simulink model "tst4"  (R2024b)
settings: Solver=ode45  StartTime=0.0  StopTime=100  FixedStep=0.1  RelTol=1e-3  EnableMultiTasking=on
Description:
  | Simulating Automatic Climate Control Systems
  | 
  | This example shows how to use Simulink(R) and Stateflow(R) to simulate the working of
  | an automatic climate control system in a car. You can enter a temperature
  | value you would like the air in the car to reach by double clicking the
  | User Setpoint in Celsius Block and entering the temperature value. You can
  | also set the External Temperature in Celsius in a similar way. The
  | numerical display on the right-hand side of the model shows the reading
  | of a temperature sensor placed behind the driver's head. This is the
  | temperature that the driver should be feeling. When the model is run and
  | the climate control is active, it is this display box whose value changes
  | to show the change of temperature in the car.
settings Model: ModifiedByFormat=The MathWorks, Inc.  Creator=The MathWorks, Inc.  LastModifiedBy=The MathWorks, Inc.
settings SolverCC: AlgebraicLoopSolver=TrustRegion  MaxZcPerStep=1
settings DataIOCC: LimitDataPoints=on  SaveFormat=Array  ReturnWorkspaceOutputs=off  SignalLoggingName=sigsOut
settings OptimizationCC: ReuseModelBlockBuffer=off  ExpressionDepthLimit=2147483647  InitFltsAndDblsToZero=on  LifeSpan=inf
settings DebuggingCC: SaveWithParameterizedLinksMsg=none  SignalResolutionControl=TryResolveAllWithWarning  MultiTaskDSMMsg=warning  MultiTaskCondExecSysMsg=none  SigSpecEnsureSampleTimeMsg=none  FcnCallInpInsideContextMsg=warning  UnconnectedInputMsg=warning  UnconnectedOutputMsg=warning  UnconnectedLineMsg=warning  StateNameClashWarn=warning  SFUnexpectedBacktrackingDiag=warning  SFNoUnconditionalDefaultTransitionDiag=warning  SFExecutionAtInitializationDiag=none  ArithmeticOperatorsInVariantConditions=warning
settings HardwareCC: ProdBitPerPointer=32  ProdBitPerSizeT=32  ProdBitPerPtrDiffT=32  ProdLargestAtomicFloat=None  ProdIntDivRoundTo=Undefined  ProdEndianess=Unspecified  ProdWordSize=32  ProdHWDeviceType=32-bit Generic
settings ModelReferenceCC: EnableRefExpFcnMdlSchedulingChecks=on  PropagateSignalLabelsOutOfModel=off
settings SFSimCC: SimUseLocalCustomCode=off  SimParseCustomCode=off  CustomCodeUndefinedFunction=UseInterfaceOnly
settings RTWCC: RTWUseLocalCustomCode=off  GPUComputeCapability=3.5  DLArmComputeVersion=19.05
settings CodeAppCC: StateflowObjectComments=on
settings GRTTargetCC: TargetFcnLib=ansi_tfl_tmw.mat  TargetLangStandard=C89/C90 (ANSI)  CombineOutputUpdateFcns=off  GRTInterface=on
settings ConfigComp: CovMetricSettings=dw  CovSaveCumulativeToWorkspaceVar=on  CovSaveSingleToWorkspaceVar=on  CovExternalEMLEnable=off  CovSFcnEnable=off

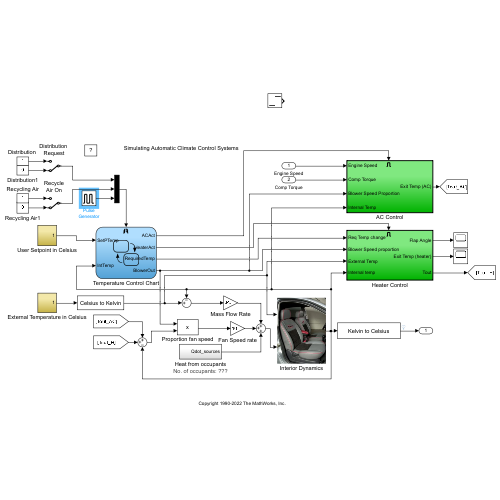
[thumbnail: Simulink's stored preview of the top-level diagram]
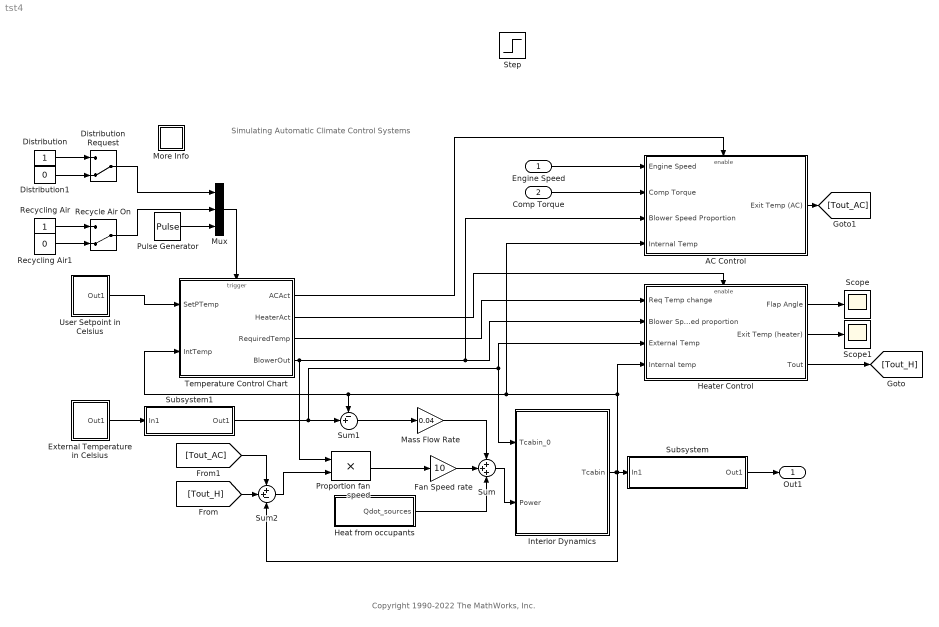
== system tst4 ==
  note: Simulating Automatic Climate Control Systems
  note: Copyright 1990-2022 The MathWorks, Inc.
  Engine Speed : Inport
  Comp Torque : Inport  Port=2
  AC Control : Subsystem  TreatAsAtomicUnit=on
  "Distribution " : Constant
  Distribution Request : ManualSwitch  CurrentSetting=0
  "Distribution1 " : Constant  Value=0
  External Temperature in Celsius : Subsystem
  Fan Speed rate : Gain  Gain=10  SaturateOnIntegerOverflow=on  OutDataTypeStr=Inherit: Same as input  ParamDataTypeStr=Inherit: Same as input
  Heat from occupants : Subsystem
      settings: AttributesFormatString=No. of occupants: %<N>
  Heater Control : Subsystem  TreatAsAtomicUnit=on
  Interior Dynamics : Subsystem  mask(Vehicle Cabin Dynamics){}
      mask Display: image('$imagefile'); % Use "Edit Image" on toolstrip to change.
  Mass Flow Rate : Gain  Gain=0.04  SaturateOnIntegerOverflow=on  OutDataTypeStr=Inherit: Same as input  ParamDataTypeStr=Inherit: Same as input
  More Info : Subsystem
      settings: OpenFcn=showExample('simulink_automotive/SimulatingAutomaticClimateControlSystemsExample')
      mask Display: disp('?')
  Mux : Mux  Inputs=3
  Proportion fan speed : Product  InputSameDT=on  SaturateOnIntegerOverflow=on  OutDataTypeStr=Inherit: Same as first input
  Pulse Generator : DiscretePulseGenerator  PulseType=Time based  Period=1/60  PulseWidth=50
  Recycle Air On : ManualSwitch  CurrentSetting=0
  Recycling Air : Constant
  Recycling Air1 : Constant  Value=0
  Scope : Scope
  Scope1 : Scope
  Step : Step  SampleTime=0
  Subsystem : Subsystem
      mask Display: disp('Kelvin to Celsius')
  Subsystem1 : Subsystem
      mask Display: disp('Celsius to Kelvin')
  Sum : Sum  Inputs=+++  InputSameDT=on  SaturateOnIntegerOverflow=on  OutDataTypeStr=Inherit: Same as first input
  Sum1 : Sum  Inputs=-+|  InputSameDT=on  SaturateOnIntegerOverflow=on  OutDataTypeStr=Inherit: Same as first input
  Sum2 : Sum  Inputs=++-  InputSameDT=on  SaturateOnIntegerOverflow=on  OutDataTypeStr=Inherit: Same as first input
  Temperature Control Chart : Stateflow chart  TreatAsAtomicUnit=on
  User Setpoint in Celsius : Subsystem
  Out1 : Outport
  wires:
  "Distribution "/1 -> Distribution Request/1
  "Distribution1 "/1 -> Distribution Request/2
  Recycling Air1/1 -> Recycle Air On/2
  User Setpoint in Celsius/1(Out1) -> Temperature Control Chart/1(SetPTemp)
  Recycling Air/1 -> Recycle Air On/1
  Interior Dynamics/1("Tcabin ") -> Sum2/3, Heater Control/4(Internal temp), AC Control/4(Internal Temp), Sum1/1, Temperature Control Chart/2(IntTemp), Subsystem/1(In1)
  Subsystem/1(Out1) -> Out1/1
  External Temperature in Celsius/1(Out1) -> Subsystem1/1(In1)
  Mass Flow Rate/1 -> Sum/1
  Sum1/1 -> Mass Flow Rate/1
  Subsystem1/1(Out1) -> Sum1/2, Interior Dynamics/1(Tcabin_0), Heater Control/3(External Temp)
  Sum2/1 -> Proportion fan speed/2
  Temperature Control Chart/4(BlowerOut) -> AC Control/3(Blower Speed Proportion), Heater Control/2(Blower Speed proportion), Proportion fan speed/1
  Proportion fan speed/1 -> Fan Speed rate/1
  Temperature Control Chart/2(" HeaterAct") -> Heater Control/Enable
  Heater Control/3(Tout) -> [Tout_H]
  [Tout_H] -> Sum2/2
  Temperature Control Chart/1(" ACAct") -> AC Control/Enable
  [Tout_AC] -> Sum2/1
  Temperature Control Chart/3(RequiredTemp) -> Heater Control/1(Req Temp change)
  AC Control/1(Exit Temp (AC)) -> [Tout_AC]
  Mux/1 -> Temperature Control Chart/Trigger
  Sum/1 -> Interior Dynamics/2(Power)
  Recycle Air On/1 -> Mux/2
  Distribution Request/1 -> Mux/1
  Fan Speed rate/1 -> Sum/2
  Heat from occupants/1(Qdot_sources) -> Sum/3
  Heater Control/1(Flap Angle) -> Scope/1
  Heater Control/2(Exit Temp (heater)) -> Scope1/1
  Engine Speed/1 -> AC Control/1(Engine Speed)
  Comp Torque/1 -> AC Control/2(Comp Torque)
  Pulse Generator/1 -> Mux/3

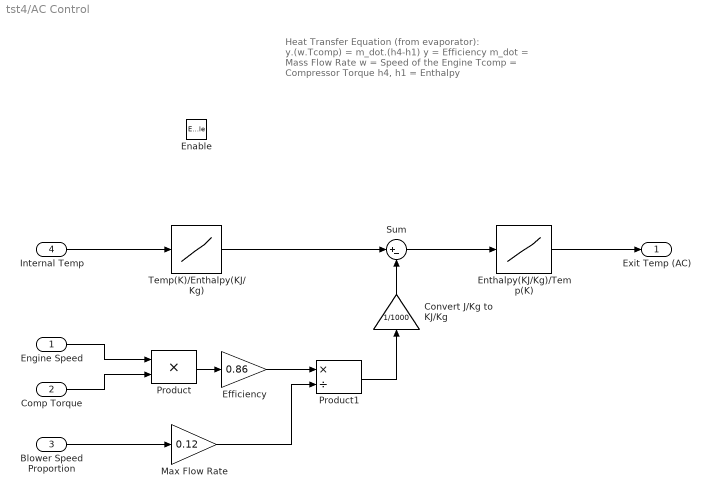
== system tst4/AC Control ==
  note: Heat Transfer Equation (from evaporator):
      |
      | y.(w.Tcomp) = m_dot.(h4-h1)
      |
      |          y = Efficiency
      |  m_dot = Mass Flow Rate
      | 	  w = Speed of the Engine
      | Tcomp = Compressor Torque
      |  h4, h1 = Enthalpy
  Engine Speed : Inport
  Comp Torque : Inport  Port=2
  Blower Speed Proportion : Inport  Port=3
  Internal Temp : Inport  Port=4
  Enable : EnablePort  StatesWhenEnabling=reset  PropagateVarSize=During execution  ZeroCross=off
  Convert J/Kg to KJ/Kg : Gain  Gain=1/1000
  Efficiency : Gain  Gain=0.86  SaturateOnIntegerOverflow=on  OutDataTypeStr=Inherit: Same as input  ParamDataTypeStr=Inherit: Same as input
  Enthalpy(KJ/Kg)/Temp(K) : Lookup_n-D  NumberOfTableDimensions=1  BreakpointsForDimension1=[ 219.97 230.02 240.02 250.05 260.09 270.11 280.13 285.14 290.16 295.17 300.19 305.22 310.24 315.27 320.29]  Table=[220 230 240 250 260 270 280 285 290 295 300 305 310 315 320]  SaturateOnIntegerOverflow=on
  Max Flow Rate : Gain  Gain=0.12  SaturateOnIntegerOverflow=on  OutDataTypeStr=Inherit: Same as input  ParamDataTypeStr=Inherit: Same as input
  Product : Product  InputSameDT=on  SaturateOnIntegerOverflow=on  OutDataTypeStr=Inherit: Same as first input
  Product1 : Product  Inputs=*/  InputSameDT=on  SaturateOnIntegerOverflow=on  OutDataTypeStr=Inherit: Same as first input
  Sum : Sum  Inputs=|+-  InputSameDT=on  SaturateOnIntegerOverflow=on  OutDataTypeStr=Inherit: Same as first input
  Temp(K)/Enthalpy(KJ/Kg) : Lookup_n-D  NumberOfTableDimensions=1  BreakpointsForDimension1=[220 230 240 250 260 270 280 285 290 295 300 305 310 315 320]  Table=[219.97 230.02 240.02 250.05 260.09 270.11 280.13 285.14 290.16 295.17 300.19 305.22 310.24 315.27 320.29]  SaturateOnIntegerOverflow=on
  Exit Temp (AC) : Outport  OutputWhenDisabled=reset  InitialOutput=0  VectorParamsAs1DForOutWhenUnconnected=off
  wires:
  Sum/1 -> Enthalpy(KJ/Kg)/Temp(K)/1
  Product1/1 -> Convert J/Kg to KJ/Kg/1
  Temp(K)/Enthalpy(KJ/Kg)/1 -> Sum/1
  Internal Temp/1 -> Temp(K)/Enthalpy(KJ/Kg)/1
  Max Flow Rate/1 -> Product1/2
  Blower Speed Proportion/1 -> Max Flow Rate/1
  Efficiency/1 -> Product1/1
  Product/1 -> Efficiency/1
  Comp Torque/1 -> Product/2
  Engine Speed/1 -> Product/1
  Enthalpy(KJ/Kg)/Temp(K)/1 -> Exit Temp (AC)/1
  Convert J/Kg to KJ/Kg/1 -> Sum/2

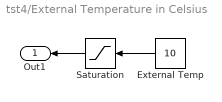
== system tst4/External Temperature in Celsius ==
  External Temp : Constant  Value=10
  Saturation : Saturate  UpperLimit=100  LowerLimit=-99
  Out1 : Outport  VectorParamsAs1DForOutWhenUnconnected=off
  wires:
  External Temp/1 -> Saturation/1
  Saturation/1 -> Out1/1

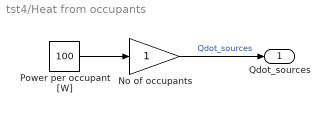
== system tst4/Heat from occupants ==
  No of occupants : Gain  SaturateOnIntegerOverflow=on  OutDataTypeStr=Inherit: Same as input  ParamDataTypeStr=Inherit: Same as input
  Power per occupant [W] : Constant  Value=100
  Qdot_sources : Outport  VectorParamsAs1DForOutWhenUnconnected=off
  wires:
  Power per occupant [W]/1 -> No of occupants/1
  No of occupants/1 -> Qdot_sources/1  "Qdot_sources"

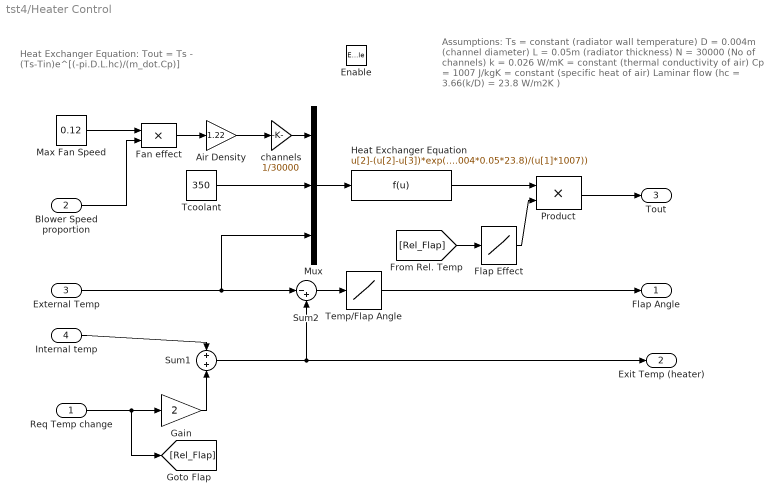
== system tst4/Heater Control ==
  note: Assumptions:
      | Ts = constant (radiator wall temperature)
      | D = 0.004m (channel diameter)
      | L = 0.05m (radiator thickness)
      | N = 30000 (No of channels)
      | k = 0.026 W/mK = constant (thermal conductivity of air)
      | Cp = 1007 J/kgK = constant (specific heat of air)
      | Laminar flow (hc = 3.66(k/D) = 23.8 W/m2K )
  note: Heat Exchanger Equation:
      | Tout = Ts - (Ts-Tin)e^[(-pi.D.L.hc)/(m_dot.Cp)]
  Req Temp change : Inport
  Blower Speed proportion : Inport  Port=2
  External Temp : Inport  Port=3
  Internal temp : Inport  Port=4
  Enable : EnablePort  StatesWhenEnabling=reset  PropagateVarSize=During execution  ZeroCross=off
  Air Density : Gain  Gain=1.22  SaturateOnIntegerOverflow=on  OutDataTypeStr=Inherit: Same as input  ParamDataTypeStr=Inherit: Same as input
  Fan effect : Product  InputSameDT=on  SaturateOnIntegerOverflow=on  OutDataTypeStr=Inherit: Same as first input
  Flap Effect : Lookup_n-D  NumberOfTableDimensions=1  BreakpointsForDimension1="[0 3 5 10 50  90 100 200 ]"  Table="[0 300 100  10 10  10 3 1]"  SaturateOnIntegerOverflow=on
  Gain : Gain  Gain=2  SaturateOnIntegerOverflow=on  OutDataTypeStr=Inherit: Same as input  ParamDataTypeStr=Inherit: Same as input
  Heat Exchanger Equation : Fcn  Expr=u[2]-(u[2]-u[3])*exp(-(pi*0.004*0.05*23.8)/(u[1]*1007))
  Max Fan Speed : Constant  Value=0.12
  Mux : Mux  Inputs=3
  Product : Product  InputSameDT=on  SaturateOnIntegerOverflow=on  OutDataTypeStr=Inherit: Same as first input
  Sum1 : Sum  InputSameDT=on  SaturateOnIntegerOverflow=on  OutDataTypeStr=Inherit: Same as first input
  Sum2 : Sum  Inputs=|-+  InputSameDT=on  SaturateOnIntegerOverflow=on  OutDataTypeStr=Inherit: Same as first input
  "Tcoolant " : Constant  Value=350
  Temp/Flap Angle : Lookup_n-D  NumberOfTableDimensions=1  BreakpointsForDimension1=[0 10 20 30 40 50 60 75 100 200]  Table=[0 20 30 45 60 75 90 90 90 90]  SaturateOnIntegerOverflow=on
  channels : Gain  Gain=1/30000  SaturateOnIntegerOverflow=on  OutDataTypeStr=Inherit: Same as input  ParamDataTypeStr=Inherit: Same as input
  Flap Angle : Outport  OutputWhenDisabled=reset  InitialOutput=0  VectorParamsAs1DForOutWhenUnconnected=off
  Exit Temp (heater) : Outport  Port=2  OutputWhenDisabled=reset  InitialOutput=0  VectorParamsAs1DForOutWhenUnconnected=off
  Tout : Outport  Port=3  OutputWhenDisabled=reset  InitialOutput=0  VectorParamsAs1DForOutWhenUnconnected=off
  wires:
  Heat Exchanger Equation/1 -> Product/1
  External Temp/1 -> Mux/3, Sum2/1
  Blower Speed proportion/1 -> Fan effect/2
  Max Fan Speed/1 -> Fan effect/1
  Fan effect/1 -> Air Density/1
  Mux/1 -> Heat Exchanger Equation/1
  Air Density/1 -> channels/1
  channels/1 -> Mux/1
  "Tcoolant "/1 -> Mux/2
  Flap Effect/1 -> Product/2
  Product/1 -> Tout/1
  Temp/Flap Angle/1 -> Flap Angle/1
  Sum2/1 -> Temp/Flap Angle/1
  Internal temp/1 -> Sum1/1
  Gain/1 -> Sum1/2
  Sum1/1 -> Exit Temp (heater)/1, Sum2/2
  Req Temp change/1 -> Gain/1, [Rel_Flap]
  [Rel_Flap] -> Flap Effect/1

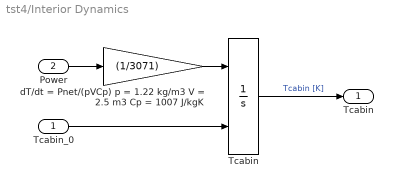
== system tst4/Interior Dynamics ==
  Tcabin_0 : Inport
  Power : Inport  Port=2
  Tcabin : Integrator  InitialConditionSource=external  InitialCondition=291  ZeroCross=off
  dT/dt = Pnet/(pVCp) p = 1.22 kg/m3 V = 2.5 m3 Cp = 1007 J/kgK : Gain  Gain=(1/3071)  SaturateOnIntegerOverflow=on  OutDataTypeStr=Inherit: Same as input  ParamDataTypeStr=Inherit: Same as input
  "Tcabin " : Outport  VectorParamsAs1DForOutWhenUnconnected=off
  wires:
  dT/dt = Pnet/(pVCp) p = 1.22 kg/m3 V = 2.5 m3 Cp = 1007 J/kgK/1 -> Tcabin/1
  Power/1 -> dT/dt = Pnet/(pVCp) p = 1.22 kg/m3 V = 2.5 m3 Cp = 1007 J/kgK/1
  Tcabin/1 -> "Tcabin "/1  "Tcabin [K]"
  Tcabin_0/1 -> Tcabin/2

== system tst4/More Info ==

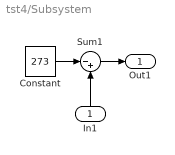
== system tst4/Subsystem ==
  In1 : Inport
  Constant : Constant  Value=273
  Sum1 : Sum  Inputs=|-+  InputSameDT=on  SaturateOnIntegerOverflow=on  OutDataTypeStr=Inherit: Same as first input
  Out1 : Outport  VectorParamsAs1DForOutWhenUnconnected=off
  wires:
  Sum1/1 -> Out1/1
  In1/1 -> Sum1/2
  Constant/1 -> Sum1/1

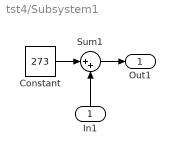
== system tst4/Subsystem1 ==
  In1 : Inport
  Constant : Constant  Value=273
  Sum1 : Sum  Inputs=|++  InputSameDT=on  SaturateOnIntegerOverflow=on  OutDataTypeStr=Inherit: Same as first input
  Out1 : Outport  VectorParamsAs1DForOutWhenUnconnected=off
  wires:
  Constant/1 -> Sum1/1
  In1/1 -> Sum1/2
  Sum1/1 -> Out1/1

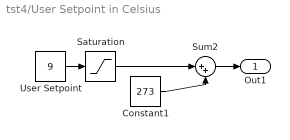
== system tst4/User Setpoint in Celsius ==
  Constant1 : Constant  Value=273
  Saturation : Saturate  UpperLimit=100  LowerLimit=-99
  Sum2 : Sum  Inputs=|++  InputSameDT=on  SaturateOnIntegerOverflow=on  OutDataTypeStr=Inherit: Same as first input
  User Setpoint : Constant  Value=9
  Out1 : Outport  VectorParamsAs1DForOutWhenUnconnected=off
  wires:
  Sum2/1 -> Out1/1
  User Setpoint/1 -> Saturation/1
  Constant1/1 -> Sum2/2
  Saturation/1 -> Sum2/1

== stateflow chart tst4/Temperature Control Chart ==
  state Blower [parallel]
    during:setpoint_calc();
    settings: executionOrder=1
    state Blower_off
      entry:BlowerOut=0.0;
    state Blower_on
      state Blower_1
        entry:BlowerOut=0.2;
      state Blower_2
        entry:BlowerOut=0.4;
      state Blower_3
        entry:BlowerOut=0.6;
      state Blower_4
        entry:BlowerOut=0.8;
      state Blower_5
        entry:BlowerOut=1.0;
      (default) -> Blower_1
      Blower_on -> Blower_1 [order 5] : E[~in(Blower_1) && in_temp_range(1.5,5)]
      Blower_on -> Blower_2 [order 4] : E[~in(Blower_2) && in_temp_range(7,10)]
      Blower_on -> Blower_3 [order 3] : E[~in(Blower_3) && in_temp_range(12,15)]
      Blower_on -> Blower_4 [order 2] : E[~in(Blower_4) && in_temp_range(17,20)]
      Blower_on -> Blower_5 [order 1] : E[~in(Blower_5) && in_temp_range(22,200)]
    state setpoint_calc() [function]
      (default) -> (junction 51) : {RequiredTemp = SetPTemp-IntTemp;}
      (junction 51) -> (junction 48) [order 1] : [RequiredTemp<0.0]
          | {absTempDiff = -RequiredTemp;}
      (junction 51) -> (junction 49) [order 2] : {absTempDiff = RequiredTemp;}
    state b = in_temp_range(minTemp,maxTemp) [function]
      (default) -> (junction 50) : {b = (absTempDiff>minTemp) &&  ...
          |         (absTempDiff<maxTemp);}
    (default) -> Blower_off
    Blower_off -> Blower_on : E[in_temp_range(.5,203)]
    Blower_on -> Blower_off [order 1] : E[absTempDiff>203 || absTempDiff<=0.5]
  state Heater_AC [parallel]
    settings: executionOrder=2
    state H_offAC_off
    state ACAct
    state HeaterAct
    ACAct -> H_offAC_off : E[SetPTemp-IntTemp>=-0.5]
    HeaterAct -> H_offAC_off : E[SetPTemp-IntTemp<=0.5]
    H_offAC_off -> HeaterAct [order 2] : E[SetPTemp-IntTemp>0.5]
    H_offAC_off -> ACAct [order 1] : E[SetPTemp-IntTemp<-0.5]
    (default) -> H_offAC_off
  state AirDist [parallel]
    settings: executionOrder=3
    state Feet
    state Face
    state Defrost
    (default) -> Face
    Feet -> Defrost : DistReq
    Face -> Feet : DistReq
    Defrost -> Face : DistReq
  state Recyc_Air [parallel]
    settings: executionOrder=4
    state Recyc_on
    state Recyc_off
    (default) -> Recyc_on
    Recyc_on -> Recyc_off [order 2] : RecycReq
    Recyc_off -> Recyc_on : RecycReq
    Recyc_on -> Recyc_off [order 1] : en(AirDist.Defrost)
  data: minTemp function_input double; b function_output boolean; maxTemp function_input double; ACAct output boolean; SetPTemp input double; IntTemp input double; HeaterAct output boolean; RequiredTemp output double; BlowerOut output double; absTempDiff local double
  events: DistReq input EITHER_EDGE_EVENT; RecycReq input EITHER_EDGE_EVENT; E input EITHER_EDGE_EVENT
